simulink model "cbf_control"  (R2024b)
settings: Solver=VariableStepAuto  StartTime=0.0  StopTime=10.0  RelTol=1e-3
settings Model: Creator=tatiana  LastModifiedBy=tatiana

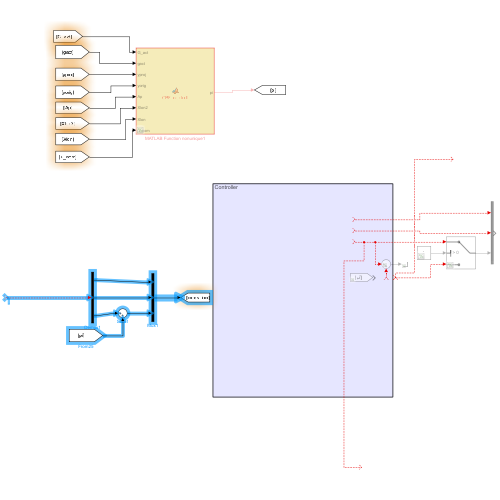
[thumbnail: Simulink's stored preview of the top-level diagram]
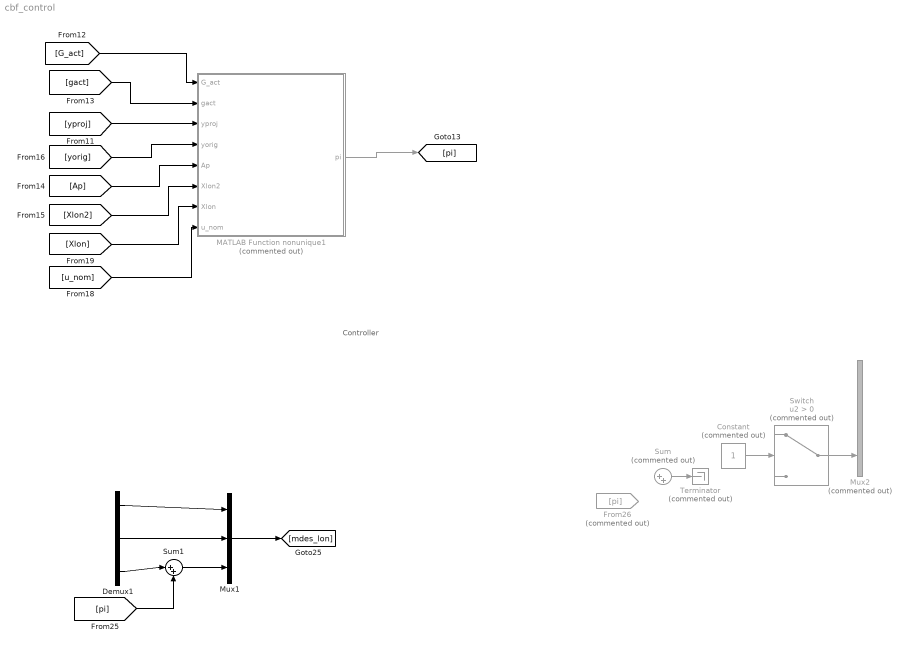
== system cbf_control ==
  note: Controller
  Constant : Constant  Commented=on
  Demux1 : Demux  Outputs=3
  From26 : From  Commented=on  GotoTag=pi
  MATLAB Function nonunique1 : MATLAB Function  Commented=on  TreatAsAtomicUnit=on
  Mux1 : Mux  Inputs=3
  Mux2 : Mux  Commented=on  Inputs=3
  Sum : Sum  Commented=on  Inputs=|++
  Sum1 : Sum  Inputs=|++
  Switch : Switch  Commented=on  Criteria=u2 > Threshold  SaturateOnIntegerOverflow=off  InputSameDT=off
  Terminator : Terminator  Commented=on
  wires:
  MATLAB Function nonunique1/1(pi) -> [pi]
  [yorig] -> MATLAB Function nonunique1/4(yorig)
  [yproj] -> MATLAB Function nonunique1/3(yproj)
  [Ap] -> MATLAB Function nonunique1/5(Ap)
  [G_act] -> MATLAB Function nonunique1/1(G_act)
  [Xlon2] -> MATLAB Function nonunique1/6(Xlon2)
  [u_nom] -> MATLAB Function nonunique1/8(u_nom)
  [gact] -> MATLAB Function nonunique1/2(gact)
  [Xlon] -> MATLAB Function nonunique1/7(Xlon)
  Sum/1 -> Terminator/1
  ? -> Mux2/1
  ? -> Switch/1, Sum/1
  ? -> ?
  ? -> Mux2/2
  ? -> Sum/2
  Constant/1 -> Switch/2
  ? -> Switch/3
  Switch/1 -> Mux2/3
  Demux1/3 -> Sum1/1
  ? -> Demux1/1
  [pi] -> Sum1/2
  Demux1/2 -> Mux1/2
  Demux1/1 -> Mux1/1
  Sum1/1 -> Mux1/3
  Mux1/1 -> [mdes_lon]

== matlab function cbf_control/MATLAB Function nonunique1 ==
  data: G_act input; pi output; gact input; yproj input; yorig input; Ap input; Xlon2 input; Xlon input; u_nom input
function pi  = CBF_control(G_act, gact, yproj, yorig, Ap, Xlon2, Xlon, u_nom)

% Initialize active constraints at every time step

% Q = eye(2);  
% 
% M = inv(G_act*inv(Q)*inv(Q)'*G_act');
% 
% Gbar = inv(Q)*inv(Q)'*G_act'*M*G_act;
% 
% gbar = inv(Q)*inv(Q)'*G_act'*M*gact;
%
% yproj =[q;theta]
% yorig =[q;theta]


% Initialize control augmentation
pi = 0;

% Check whether either theta or q was projected
tol = 1e-10;

if norm(yorig-yproj) <= tol
    pi = 0;
    return
end

    % Initialize outputs
    Gbar = zeros(2,2);
    gbar = zeros(2,1);
    
    % Calculate denominator
    M = G_act*G_act';
    
    % Only calculate when constraint is active
    if M > 1e-12
    
        Gbar = (G_act'*G_act)/M;
    
        gbar = (G_act'*gact)/M;
    
    end
    
    Mu_Jy = Ap(3,1);
    Mw_Jy = Ap(3,2);
    Mq_Jy = Ap(3,3);
    
    %u = Xlon2(1); w = Xlon2(2); q = Xlon2(3);
    u = Xlon(1); w = Xlon(2); q = Xlon(3);
    
    %Delta_y = Gbar*y-gbar
    %h_1 = 0.5*Delta_y^T*Delta_yq-0.5R^2
    % H_1(y)=(Gbar*y-gbar)'*Gbar*ydot + alpha_0*h_1(y) <= 0;
    %H_1(y)= a * Gbar  *ydot + alpha_0*h_1(y) <= 0
    %ydot = [fq; q] + [1; 0]*pi
    By = [1; 0];
    %fy = [fq; q];
    %H_1(y)= a * Gbar  *(fy+By*pi)+ alpha_0*h_1(y) <= 0
    % a'*Gbar*By*pi <= -a'*Gbar*fy-alpha_0*h_1
    
    % Parameters
    R=0.1;
    alpha_0 = 0.1
    
    % From projection 
    deltay = (Gbar*yorig-gbar);
    %y_q_dot = fq(x) + pi;
    %fq(x) = Mu_Jy*u + Mw_Jy*w + Mq_Jy*q;
    
    %ydot = [fq; q] + [1; 0]*pi
    fq = Ap(3,1:3)*Xlon2;
    fy = [fq; q];
    h_1 = (0.5*deltay'*deltay)-(0.5*R^2);
    tau_1 = -(deltay'*Gbar*fy) - (alpha_0*h_1);
    hu1 = deltay'*Gbar*By  % is a scalar so no need for inverse
    pi = tau_1/hu1;

    % u = u_nom - P^{-1}\gamma(x)*max{0,\frac{-\tau(x)+\gamma(x)^T u_nom}{\gamma(x)^T P^{-1}\gamma(x)}
    % u = u_nom - P^{-1}*hu1*max{0,(-\tau_1 + hu1^T * u_nom) / hu1^T * P^{-1} * hu1)
    P = 1;
    k = -tau_1+(hu1'*u_nom);
    pi = ((inv(P)*hu1)/(hu1'*inv(P)*hu1))*max(0,k);


end
